simulink model "s_b8a4x128f"  (R2016b)
settings: Solver=VariableStepDiscrete  StartTime=0.0  StopTime=1  RelTol=1e-3
undefined symbols (not defined in the file): fft_stages, n_bits_ants, n_bits_xengs
libraries: xbsIndex_r4 x21069, casper_library_misc x164, casper_library_scopes x9, xbsReplacements_r4 x9, casper_library_delays x8, xps_library x3
(part 29 of 186)

== system s_b8a4x128f/sys1/x_cast ==
  in : Inport
  Concat : xbsIndex_r4/Concat  num_inputs=8  dbl_ovrd=off  block_type=concat
      settings: block_version=9.2.01
  Convert{,1..7} (8 alike) : xbsIndex_r4/Convert  gui_display_data_type=Fixed-point  arith_type="Signed  (2's comp)"  n_bits=n_bits_out  bin_pt=fix_pnt_pos  float_type=Single  exp_bits=8  fraction_bits=24  quantization=Truncate  overflow=Wrap  en=off  latency=0  pipeline=off  dbl_ovrd=off  block_type=convert
      settings: block_version=10.1.3
  Slice : xbsIndex_r4/Slice  nbits=n_bits_in  boolean_output=off  mode=Lower Bit Location + Width  bit1=0  base1=MSB of Input  bit0=bit_offsets(1)*n_bits_in  base0=LSB of Input  dbl_ovrd=off  block_type=slice
      settings: infoedit="Extracts a given range of bits from each input sample and presents it at the output.  The output type is ordinarily unsigned with binary point at zero, but can be Boolean when the slice is one bit wide.<P><P>Hardware notes: In hardware this block costs nothing."  block_version=10.1.3
  Slice1 : xbsIndex_r4/Slice  nbits=n_bits_in  boolean_output=off  mode=Lower Bit Location + Width  bit1=0  base1=MSB of Input  bit0=bit_offsets(2)*n_bits_in  base0=LSB of Input  dbl_ovrd=off  block_type=slice
      settings: infoedit="Extracts a given range of bits from each input sample and presents it at the output.  The output type is ordinarily unsigned with binary point at zero, but can be Boolean when the slice is one bit wide.<P><P>Hardware notes: In hardware this block costs nothing."  block_version=10.1.3
  Slice2 : xbsIndex_r4/Slice  nbits=n_bits_in  boolean_output=off  mode=Lower Bit Location + Width  bit1=0  base1=MSB of Input  bit0=bit_offsets(3)*n_bits_in  base0=LSB of Input  dbl_ovrd=off  block_type=slice
      settings: infoedit="Extracts a given range of bits from each input sample and presents it at the output.  The output type is ordinarily unsigned with binary point at zero, but can be Boolean when the slice is one bit wide.<P><P>Hardware notes: In hardware this block costs nothing."  block_version=10.1.3
  Slice3 : xbsIndex_r4/Slice  nbits=n_bits_in  boolean_output=off  mode=Lower Bit Location + Width  bit1=0  base1=MSB of Input  bit0=bit_offsets(4)*n_bits_in  base0=LSB of Input  dbl_ovrd=off  block_type=slice
      settings: infoedit="Extracts a given range of bits from each input sample and presents it at the output.  The output type is ordinarily unsigned with binary point at zero, but can be Boolean when the slice is one bit wide.<P><P>Hardware notes: In hardware this block costs nothing."  block_version=10.1.3
  Slice4 : xbsIndex_r4/Slice  nbits=n_bits_in  boolean_output=off  mode=Lower Bit Location + Width  bit1=0  base1=MSB of Input  bit0=bit_offsets(5)*n_bits_in  base0=LSB of Input  dbl_ovrd=off  block_type=slice
      settings: infoedit="Extracts a given range of bits from each input sample and presents it at the output.  The output type is ordinarily unsigned with binary point at zero, but can be Boolean when the slice is one bit wide.<P><P>Hardware notes: In hardware this block costs nothing."  block_version=10.1.3
  Slice5 : xbsIndex_r4/Slice  nbits=n_bits_in  boolean_output=off  mode=Lower Bit Location + Width  bit1=0  base1=MSB of Input  bit0=bit_offsets(6)*n_bits_in  base0=LSB of Input  dbl_ovrd=off  block_type=slice
      settings: infoedit="Extracts a given range of bits from each input sample and presents it at the output.  The output type is ordinarily unsigned with binary point at zero, but can be Boolean when the slice is one bit wide.<P><P>Hardware notes: In hardware this block costs nothing."  block_version=10.1.3
  Slice6 : xbsIndex_r4/Slice  nbits=n_bits_in  boolean_output=off  mode=Lower Bit Location + Width  bit1=0  base1=MSB of Input  bit0=bit_offsets(7)*n_bits_in  base0=LSB of Input  dbl_ovrd=off  block_type=slice
      settings: infoedit="Extracts a given range of bits from each input sample and presents it at the output.  The output type is ordinarily unsigned with binary point at zero, but can be Boolean when the slice is one bit wide.<P><P>Hardware notes: In hardware this block costs nothing."  block_version=10.1.3
  Slice7 : xbsIndex_r4/Slice  nbits=n_bits_in  boolean_output=off  mode=Lower Bit Location + Width  bit1=0  base1=MSB of Input  bit0=bit_offsets(8)*n_bits_in  base0=LSB of Input  dbl_ovrd=off  block_type=slice
      settings: infoedit="Extracts a given range of bits from each input sample and presents it at the output.  The output type is ordinarily unsigned with binary point at zero, but can be Boolean when the slice is one bit wide.<P><P>Hardware notes: In hardware this block costs nothing."  block_version=10.1.3
  force_re{,1,4,6,8,10,12,14} (8 alike) : xbsIndex_r4/Reinterpret  force_arith_type=on  arith_type="Signed  (2's comp)"  force_bin_pt=on  bin_pt=fix_pnt_pos  block_type=reinterpret
      settings: infoedit="Changes signal type without altering the binary representation.   You can changed the signal between signed and unsigned, and relocate the binary point.<P><P>Hardware notes: In hardware this block costs nothing.<P><P>Example:  Suppose the input is 6 bits wide, signed, with 2 fractional bits, and the output is forced to unsigned with 0 fractional bits.  Then an input of -2.0 (1110.00 in binary 2's complement) becomes an output of 56 (111000 in binary)."  block_version=9.1.01
  force_re{2..3,5,7,9,11,13,15} (8 alike) : xbsIndex_r4/Reinterpret  force_arith_type=on  arith_type=Unsigned  force_bin_pt=on  bin_pt=0  block_type=reinterpret
      settings: infoedit="Changes signal type without altering the binary representation.   You can changed the signal between signed and unsigned, and relocate the binary point.<P><P>Hardware notes: In hardware this block costs nothing.<P><P>Example:  Suppose the input is 6 bits wide, signed, with 2 fractional bits, and the output is forced to unsigned with 0 fractional bits.  Then an input of -2.0 (1110.00 in binary 2's complement) becomes an output of 56 (111000 in binary)."  block_version=9.1.01
  out : Outport
  wires:
  force_re2/1 -> Concat/1
  Convert/1 -> force_re2/1
  Convert1/1 -> force_re3/1
  force_re/1 -> Convert/1
  force_re1/1 -> Convert1/1
  Slice/1 -> force_re/1
  in/1 -> Slice/1, Slice6/1, Slice7/1, Slice5/1, Slice4/1, Slice3/1, Slice2/1, Slice1/1
  Concat/1 -> out/1
  Slice1/1 -> force_re1/1
  force_re3/1 -> Concat/2
  Convert2/1 -> force_re5/1
  force_re4/1 -> Convert2/1
  Slice2/1 -> force_re4/1
  Convert3/1 -> force_re7/1
  force_re6/1 -> Convert3/1
  Slice3/1 -> force_re6/1
  Convert4/1 -> force_re9/1
  force_re8/1 -> Convert4/1
  Slice4/1 -> force_re8/1
  Convert5/1 -> force_re11/1
  force_re10/1 -> Convert5/1
  Slice5/1 -> force_re10/1
  Convert6/1 -> force_re13/1
  force_re12/1 -> Convert6/1
  Slice6/1 -> force_re12/1
  Convert7/1 -> force_re15/1
  force_re14/1 -> Convert7/1
  Slice7/1 -> force_re14/1
  force_re5/1 -> Concat/3
  force_re7/1 -> Concat/4
  force_re9/1 -> Concat/5
  force_re11/1 -> Concat/6
  force_re13/1 -> Concat/7
  force_re15/1 -> Concat/8

== system s_b8a4x128f/sys1/xeng ==
  sync_in : Inport
  ant : Inport  Port=2
  window_valid : Inport  Port=3
  mcnt_in : Inport  Port=4
  Constant : xbsIndex_r4/Constant  const=0  gui_display_data_type=Fixed-point  arith_type=Unsigned  n_bits=200  bin_pt=14  preci_type=Single  exp_width=8  frac_width=24  explicit_period=on  period=1  equ=P=C  opselect=C  inp2=PCIN>>17  opr=+  inp1=P  carry=CIN  dbl_ovrd=off  block_type=constant
  Constant1 : xbsIndex_r4/Constant  const=0  gui_display_data_type=Fixed-point  arith_type=Boolean  n_bits=1  bin_pt=14  preci_type=Single  exp_width=8  frac_width=24  explicit_period=on  period=1  equ=P=C  opselect=C  inp2=PCIN>>17  opr=+  inp1=P  carry=CIN  dbl_ovrd=off  block_type=constant
  Term1 : Terminator
  Term2 : Terminator
  Term3 : Terminator
  auto_tap : Subsystem  AncestorBlock=casper_library_correlator/auto_tap  mask(auto_tap){n_ants=8, n_simultan=2, n_bits=8, acc_len=256, add_latency=3, mult_latency=4, bram_latency=7, mult_type=1, use_bram_delay=1}
      mask prompts: n_ants "Number of antennas (total inputs = n_ants*n_simultan below)"; n_simultan "Number of inputs fed-in simultaneously"; n_bits "Number of input bits (per complex component)"; acc_len "Accumulation length"; add_latency "Adder latency"; mult_latency "Multiplier latency"; bram_latency "BRAM latency"; mult_type "Multiplier Type (0=behavioural HDL, 1=embedded, 2=core)"; use_bram_delay "Implementation: Delay type (0=SLR, 1=BRAM)"
      mask init:
      | fix_pnt_pos = (n_bits-1)*2;
      | bit_growth = ceil(log2(acc_len));
      | ant_bits = ceil(log2(n_ants));
      | n_bits_out = (2*n_bits + 1 + bit_growth);
      | 
      | params = get_mask_params(gcb);
      | auto_tap_init(gcb, params{:});
      settings: AttributesFormatString=mult_typ=1, del_typ=1
  baseline_tap1 : Subsystem  AncestorBlock=casper_library_correlator/baseline_tap  mask(baseline_tap){n_ants=8, ant_sep=1, n_bits=8, acc_len=256, add_latency=3, mult_latency=4, bram_latency=7, mult_type=1, use_bram_delay=1}
      mask prompts: n_ants "Number of antennas"; ant_sep "Antenna Seperation"; n_bits "number of input bits (per complex component)"; acc_len "accumulation length"; add_latency "Adder latency"; mult_latency "Multiplier latency"; bram_latency "BRAM latency"; mult_type "Multiplier Type (0=behavioural HDL, 1=embedded, 2=core)"; use_bram_delay "Use BRAM delays"
      mask init: same as s_b8a4x128f/sys0/xeng/baseline_tap1
      settings: AttributesFormatString=ant_sep=1, mult=1, bram=1
  baseline_tap2 : Subsystem  AncestorBlock=casper_library_correlator/baseline_tap  mask(baseline_tap){n_ants=8, ant_sep=2, n_bits=8, acc_len=256, add_latency=3, mult_latency=4, bram_latency=7, mult_type=1, use_bram_delay=1}
      mask prompts: n_ants "Number of antennas"; ant_sep "Antenna Seperation"; n_bits "number of input bits (per complex component)"; acc_len "accumulation length"; add_latency "Adder latency"; mult_latency "Multiplier latency"; bram_latency "BRAM latency"; mult_type "Multiplier Type (0=behavioural HDL, 1=embedded, 2=core)"; use_bram_delay "Use BRAM delays"
      mask init: same as s_b8a4x128f/sys0/xeng/baseline_tap1
      settings: AttributesFormatString=ant_sep=2, mult=1, bram=1
  baseline_tap3 : Subsystem  AncestorBlock=casper_library_correlator/baseline_tap  mask(baseline_tap){n_ants=8, ant_sep=3, n_bits=8, acc_len=256, add_latency=3, mult_latency=4, bram_latency=7, mult_type=1, use_bram_delay=1}
      mask prompts: n_ants "Number of antennas"; ant_sep "Antenna Seperation"; n_bits "number of input bits (per complex component)"; acc_len "accumulation length"; add_latency "Adder latency"; mult_latency "Multiplier latency"; bram_latency "BRAM latency"; mult_type "Multiplier Type (0=behavioural HDL, 1=embedded, 2=core)"; use_bram_delay "Use BRAM delays"
      mask init: same as s_b8a4x128f/sys0/xeng/baseline_tap1
      settings: AttributesFormatString=ant_sep=3, mult=1, bram=1
  baseline_tap4 : Subsystem  AncestorBlock=casper_library_correlator/baseline_tap  mask(baseline_tap){n_ants=8, ant_sep=4, n_bits=8, acc_len=256, add_latency=3, mult_latency=4, bram_latency=7, mult_type=1, use_bram_delay=1}
      mask prompts: n_ants "Number of antennas"; ant_sep "Antenna Seperation"; n_bits "number of input bits (per complex component)"; acc_len "accumulation length"; add_latency "Adder latency"; mult_latency "Multiplier latency"; bram_latency "BRAM latency"; mult_type "Multiplier Type (0=behavioural HDL, 1=embedded, 2=core)"; use_bram_delay "Use BRAM delays"
      mask init: same as s_b8a4x128f/sys0/xeng/baseline_tap1
      settings: AttributesFormatString=ant_sep=4, mult=1, bram=1
  delay : xbsIndex_r4/Delay  rst=off  infoeditControl=Selection of Reset will increase slice count due to use of real FFs and instead of SRLs  en=off  latency=1  reg_retiming=on  dbl_ovrd=off  block_type=delay
  sample_and_hold1 : Subsystem  AncestorBlock=casper_library_misc/sample_and_hold  mask(sample_and_hold){period=2048}
      mask prompts: period "Sample period (clocks)"
      mask help: This block will sample an input signal at a user specified rate and hold the value on the output.
  sample_and_hold2 : Subsystem  AncestorBlock=casper_library_misc/sample_and_hold  mask(sample_and_hold){period=2048}
      mask prompts: period "Sample period (clocks)"
      mask help: This block will sample an input signal at a user specified rate and hold the value on the output.
  sample_and_hold3 : Subsystem  AncestorBlock=casper_library_misc/sample_and_hold  mask(sample_and_hold){period=2048}
      mask prompts: period "Sample period (clocks)"
      mask help: This block will sample an input signal at a user specified rate and hold the value on the output.
  window_delay : casper_library_delays/window_delay  delay=269
  xeng_descramble : Subsystem  AncestorBlock=casper_library_correlator/xeng_descramble  mask(xeng_descramble){num_ants=8, n_bits=8, acc_len=256, demux_factor=1}
      mask prompts: num_ants "Number of Antennas"; n_bits "Input Bitwidth"; acc_len "X engine accumulation length"; demux_factor "Demux Factor"
      mask help:
      | NOT TESTED FOR non-2^N antennas.
      |
      | Descrambles X engine output. Optionally demuxes output.
      mask init: same as s_b8a4x128f/sys0/xeng/xeng_descramble
      settings: AttributesFormatString=num_ants=8
  sync_out : Outport
  valid : Outport  Port=2
  acc : Outport  Port=3
  mcnt_out : Outport  Port=4
  wires:
  xeng_descramble/1(acc_out) -> acc/1
  xeng_descramble/2(valid_out) -> valid/1
  xeng_descramble/3(sync_out) -> sync_out/1, sample_and_hold3/1(sync)
  baseline_tap4/4(acc_out) -> xeng_descramble/1(acc)
  baseline_tap4/5(valid_out) -> xeng_descramble/2(valid)
  baseline_tap4/7(sync_out) -> xeng_descramble/3(sync), sample_and_hold2/1(sync)
  window_delay/1 -> xeng_descramble/4(win_valid)
  ant/1 -> auto_tap/1(a_del), auto_tap/2(a_ndel)
  Constant/1 -> auto_tap/4(acc_in)
  Constant1/1 -> auto_tap/5(valid_in)
  sync_in/1 -> auto_tap/6(sync_in), sample_and_hold1/1(sync)
  window_valid/1 -> window_delay/1
  mcnt_in/1 -> sample_and_hold1/2(in)
  sample_and_hold1/1(out) -> sample_and_hold2/2(in)
  sample_and_hold2/1(out) -> sample_and_hold3/2(in)
  sample_and_hold3/1(out) -> delay/1
  delay/1 -> mcnt_out/1
  auto_tap/1(a_del_out) -> baseline_tap1/1(a_del)
  auto_tap/2(a_ndel_out) -> baseline_tap1/2(a_ndel)
  auto_tap/3(a_end_out) -> baseline_tap1/3(a_end)
  auto_tap/4(acc_out) -> baseline_tap1/4(acc_in)
  auto_tap/5(valid_out) -> baseline_tap1/5(valid_in)
  auto_tap/6(rst_out) -> baseline_tap1/6(rst)
  auto_tap/7(sync_out) -> baseline_tap1/7(sync1)
  baseline_tap1/1(a_del_out) -> baseline_tap2/1(a_del)
  baseline_tap1/2(a_ndel_out) -> baseline_tap2/2(a_ndel)
  baseline_tap1/3(a_end_out) -> baseline_tap2/3(a_end)
  baseline_tap1/4(acc_out) -> baseline_tap2/4(acc_in)
  baseline_tap1/5(valid_out) -> baseline_tap2/5(valid_in)
  baseline_tap1/6(rst_out) -> baseline_tap2/6(rst)
  baseline_tap1/7(sync_out) -> baseline_tap2/7(sync1)
  baseline_tap2/1(a_del_out) -> baseline_tap3/1(a_del)
  baseline_tap2/2(a_ndel_out) -> baseline_tap3/2(a_ndel)
  baseline_tap2/3(a_end_out) -> baseline_tap3/3(a_end)
  baseline_tap2/4(acc_out) -> baseline_tap3/4(acc_in)
  baseline_tap2/5(valid_out) -> baseline_tap3/5(valid_in)
  baseline_tap2/6(rst_out) -> baseline_tap3/6(rst)
  baseline_tap2/7(sync_out) -> baseline_tap3/7(sync1)
  baseline_tap3/1(a_del_out) -> baseline_tap4/1(a_del)
  baseline_tap3/2(a_ndel_out) -> baseline_tap4/2(a_ndel)
  baseline_tap3/3(a_end_out) -> baseline_tap4/3(a_end)
  baseline_tap3/4(acc_out) -> baseline_tap4/4(acc_in)
  baseline_tap3/5(valid_out) -> baseline_tap4/5(valid_in)
  baseline_tap3/6(rst_out) -> baseline_tap4/6(rst)
  baseline_tap3/7(sync_out) -> baseline_tap4/7(sync1)
  baseline_tap4/1(a_del_out) -> auto_tap/3(a_loop)
  baseline_tap4/2(a_ndel_out) -> Term1/1
  baseline_tap4/3(a_end_out) -> Term2/1
  baseline_tap4/6(rst_out) -> Term3/1

== system s_b8a4x128f/sys1/xeng_pack_out ==
  note: we must create a gap
      | between packets from
      | mutliple x-engines to allow
      | the buffers on the output switch
      | ports to drain and NIC card
      | to service the packets.
  note: if we become misaligned,
      | then we must flush the buffers
      | by reading one word, waiting "fifo_latency" clocks,
      | then reading another word until we get rb_done.
  note: the last packet
      | might be shorter!
  data_in : Inport
  valid_in : Inport  Port=2
  pkt_rdy : Inport  Port=3
  rb_done : Inport  Port=4
  timestamp : Inport  Port=5
  xeng_id : Inport  Port=6
  go : Inport  Port=7
  gap_size : Inport  Port=8
  AddSub1 : xbsIndex_r4/AddSub  mode=Subtraction  use_carryin=off  use_carryout=off  en=off  latency=1  precision=User Defined  arith_type=Unsigned  n_bits=vector_bits+1  bin_pt=0  quantization=Truncate  overflow=Saturate  use_behavioral_HDL=on  hw_selection=Fabric  pipelined=off  dbl_ovrd=off  block_type=addsub
  Concat : xbsIndex_r4/Concat  num_inputs=2  dbl_ovrd=off  block_type=concat
  Constant : xbsIndex_r4/Constant  const=0  gui_display_data_type=Boolean  arith_type=Boolean  n_bits=16  bin_pt=14  preci_type=Single  exp_width=8  frac_width=24  explicit_period=on  period=1  equ=P=C  opselect=C  inp2=PCIN>>17  opr=+  inp1=P  carry=CIN  dbl_ovrd=off  block_type=constant
  Constant1 : xbsIndex_r4/Constant  const=0  gui_display_data_type=Fixed-point  arith_type=Unsigned  n_bits=spead_lsw  bin_pt=0  preci_type=Single  exp_width=8  frac_width=24  explicit_period=on  period=1  equ=P=C  opselect=C  inp2=PCIN>>17  opr=+  inp1=P  carry=CIN  dbl_ovrd=off  block_type=constant
  Constant15 : xbsIndex_r4/Constant  const=pkt_len  gui_display_data_type=Fixed-point  arith_type=Unsigned  n_bits=vector_bits+1  bin_pt=0  preci_type=Single  exp_width=8  frac_width=24  explicit_period=on  period=1  equ=P=C  opselect=C  inp2=PCIN>>17  opr=+  inp1=P  carry=CIN  dbl_ovrd=off  block_type=constant
  Constant2 : xbsIndex_r4/Constant  const=(vector_len)-1  gui_display_data_type=Fixed-point  arith_type=Unsigned  n_bits=vector_bits+1  bin_pt=0  preci_type=Single  exp_width=8  frac_width=24  explicit_period=on  period=1  equ=P=C  opselect=C  inp2=PCIN>>17  opr=+  inp1=P  carry=CIN  dbl_ovrd=off  block_type=constant
  Constant3 : xbsIndex_r4/Constant  const=vector_len  gui_display_data_type=Fixed-point  arith_type=Unsigned  n_bits=vector_bits+1  bin_pt=0  preci_type=Single  exp_width=8  frac_width=24  explicit_period=on  period=1  equ=P=C  opselect=C  inp2=PCIN>>17  opr=+  inp1=P  carry=CIN  dbl_ovrd=off  block_type=constant
  Constant4 : xbsIndex_r4/Constant  const=0  gui_display_data_type=Boolean  arith_type=Boolean  n_bits=16  bin_pt=14  preci_type=Single  exp_width=8  frac_width=24  explicit_period=on  period=1  equ=P=C  opselect=C  inp2=PCIN>>17  opr=+  inp1=P  carry=CIN  dbl_ovrd=off  block_type=constant
  Constant6 : xbsIndex_r4/Constant  const=heap_len  gui_display_data_type=Fixed-point  arith_type=Unsigned  n_bits=spead_lsw  bin_pt=0  preci_type=Single  exp_width=8  frac_width=24  explicit_period=on  period=1  equ=P=C  opselect=C  inp2=PCIN>>17  opr=+  inp1=P  carry=CIN  dbl_ovrd=off  block_type=constant
  Constant7 : xbsIndex_r4/Constant  const=pkt_len-1  gui_display_data_type=Fixed-point  arith_type=Unsigned  n_bits=pkt_bits  bin_pt=0  preci_type=Single  exp_width=8  frac_width=24  explicit_period=on  period=1  equ=P=C  opselect=C  inp2=PCIN>>17  opr=+  inp1=P  carry=CIN  dbl_ovrd=off  block_type=constant
  Constant8 : xbsIndex_r4/Constant  const=1  gui_display_data_type=Fixed-point  arith_type=Unsigned  n_bits=ceil(log2(fifo_latency))+1  bin_pt=0  preci_type=Single  exp_width=8  frac_width=24  explicit_period=on  period=1  equ=P=C  opselect=C  inp2=PCIN>>17  opr=+  inp1=P  carry=CIN  dbl_ovrd=off  block_type=constant
  Convert{,1..4,6} (6 alike) : xbsIndex_r4/Convert  gui_display_data_type=Fixed-point  arith_type=Unsigned  n_bits=spead_lsw  bin_pt=0  float_type=Single  exp_bits=8  fraction_bits=24  quantization=Truncate  overflow=Wrap  en=off  latency=0  pipeline=off  dbl_ovrd=off  block_type=convert
      settings: block_version=11.4
  Counter1 : xbsIndex_r4/Counter  cnt_type=Free Running  cnt_to=1023  operation=Up  start_count=0  cnt_by_val=1  arith_type=Unsigned  n_bits=vector_bits+1  bin_pt=0  load_pin=off  rst=on  en=on  explicit_period=on  period=1  use_behavioral_HDL=off  implementation=Fabric  use_rpm=on  dbl_ovrd=off  block_type=counter
      settings: xl_area=[0, 0, 0, 0, 0, 0, 0]
  Delay{,3,6,10..17} (11 alike) : xbsIndex_r4/Delay  rst=off  infoeditControl=Selection of Reset will increase slice count due to use of real FFs and instead of SRLs  en=off  latency=1  reg_retiming=on  dbl_ovrd=off  block_type=delay
      settings: block_version=11.4
  Delay1 : xbsIndex_r4/Delay  rst=off  infoeditControl=Selection of Reset will increase slice count due to use of real FFs and instead of SRLs  en=on  latency=1  reg_retiming=on  dbl_ovrd=off  block_type=delay
  Delay2 : xbsIndex_r4/Delay  rst=off  infoeditControl=Selection of Reset will increase slice count due to use of real FFs and instead of SRLs  en=off  latency=fifo_latency  reg_retiming=on  dbl_ovrd=off  block_type=delay
      settings: block_version=11.4
  Delay4 : xbsIndex_r4/Delay  rst=off  infoeditControl=Selection of Reset will increase slice count due to use of real FFs and instead of SRLs  en=off  latency=fifo_latency  reg_retiming=on  dbl_ovrd=off  block_type=delay
      settings: block_version=11.4
  Delay5 : xbsIndex_r4/Delay  rst=off  infoeditControl=Selection of Reset will increase slice count due to use of real FFs and instead of SRLs  en=on  latency=1  reg_retiming=on  dbl_ovrd=off  block_type=delay
  Delay7 : xbsIndex_r4/Delay  rst=on  infoeditControl=Selection of Reset will increase slice count due to use of real FFs and instead of SRLs  en=on  latency=1  reg_retiming=on  dbl_ovrd=off  block_type=delay
  Delay8 : xbsIndex_r4/Delay  rst=on  infoeditControl=Selection of Reset will increase slice count due to use of real FFs and instead of SRLs  en=on  latency=1  reg_retiming=on  dbl_ovrd=off  block_type=delay
  Delay9 : xbsIndex_r4/Delay  rst=on  infoeditControl=Selection of Reset will increase slice count due to use of real FFs and instead of SRLs  en=on  latency=1  reg_retiming=on  dbl_ovrd=off  block_type=delay
  Gateway Out{1..21} (21 alike) : xbsIndex_r4/Gateway Out  inherit_from_input=off  hdl_port=off  rows=1  columns=1  UseAsDAC=off  DACChannel='1'  interface=None  automatic_assignment=on  address_offset=hex2dec('00')  intf_name=''  intf_description=''  timing_constraint=None  locs_specified=off  LOCs={}  io_standard={}  block_type=gatewayout
      settings: xl_area=[0, 0, 0, 0, 0, 0, 0]  block_version=10.1.3
  Inverter{1..4} (4 alike) : xbsIndex_r4/Inverter  en=off  latency=0  dbl_ovrd=off  block_type=inv
      settings: block_version=11.4
  Logical{1,3..5,13..14} (6 alike) : xbsIndex_r4/Logical  logical_function=OR  inputs=2  en=off  latency=0  precision=Full  arith_type=Unsigned  n_bits=8  bin_pt=2  align_bp=on  dbl_ovrd=off  block_type=logical
      settings: xl_area=[0, 0, 0, 0, 0, 0, 0]
  Logical{2,8..12,15} (7 alike) : xbsIndex_r4/Logical  logical_function=AND  inputs=2  en=off  latency=0  precision=Full  arith_type=Unsigned  n_bits=8  bin_pt=2  align_bp=on  dbl_ovrd=off  block_type=logical
      settings: xl_area=[0, 0, 0, 0, 0, 0, 0]
  Logical6 : xbsIndex_r4/Logical  logical_function=AND  inputs=2  en=off  latency=1  precision=Full  arith_type=Unsigned  n_bits=8  bin_pt=2  align_bp=on  dbl_ovrd=off  block_type=logical
      settings: xl_area=[0, 0, 0, 0, 0, 0, 0]
  Logical7 : xbsIndex_r4/Logical  logical_function=XOR  inputs=2  en=off  latency=0  precision=Full  arith_type=Unsigned  n_bits=8  bin_pt=2  align_bp=on  dbl_ovrd=off  block_type=logical
      settings: xl_area=[0, 0, 0, 0, 0, 0, 0]
  Mux1 : xbsIndex_r4/Mux  inputs=2  en=off  latency=1  precision=Full  arith_type="Signed  (2's comp)"  n_bits=8  bin_pt=2  quantization=Truncate  overflow=Wrap  dbl_ovrd=off  block_type=mux
      settings: xl_area=[0, 0, 0, 0, 0, 0, 0]
  Reinterpret : xbsIndex_r4/Reinterpret  force_arith_type=on  arith_type=Unsigned  force_bin_pt=on  bin_pt=0  block_type=reinterpret
      settings: infoedit="Changes signal type without altering the binary representation.   You can changed the signal between signed and unsigned, and relocate the binary point.<br><br>Hardware notes: In hardware this block costs nothing.<br><br>Example:  Suppose the input is 6 bits wide, signed, with 2 fractional bits, and the output is forced to unsigned with 0 fractional bits.  Then an input of -2.0 (1110.00 in binary 2's complement) becomes an output of 56 (111000 in binary)."
  Relational1 : xbsIndex_r4/Relational  mode=a=b  op_type=Bool  en=off  latency=0  dbl_ovrd=off  block_type=relational
      settings: xl_area=[0, 0, 0, 0, 0, 0, 0]  block_version=10.1.3
  Relational2 : xbsIndex_r4/Relational  mode=a<b  op_type=Bool  en=off  latency=0  dbl_ovrd=off  block_type=relational
      settings: xl_area=[0, 0, 0, 0, 0, 0, 0]  block_version=10.1.3
  Relational4 : xbsIndex_r4/Relational  mode=a=b  op_type=Bool  en=off  latency=0  dbl_ovrd=off  block_type=relational
      settings: xl_area=[0, 0, 0, 0, 0, 0, 0]  block_version=10.1.3
  Relational5 : xbsIndex_r4/Relational  mode=a=b  op_type=Bool  en=off  latency=0  dbl_ovrd=off  block_type=relational
      settings: xl_area=[0, 0, 0, 0, 0, 0, 0]  block_version=10.1.3
  Shift1 : xbsIndex_r4/Shift  shift_dir=Left  shift_bits=n_bits_word_size  en=off  latency=0  precision=Full  arith_type="Signed  (2's comp)"  n_bits=16  bin_pt=14  quantization=Truncate  overflow=Wrap  dbl_ovrd=off  block_type=shift
  Shift2 : xbsIndex_r4/Shift  shift_dir=Left  shift_bits=n_bits_chans  en=off  latency=0  precision=Full  arith_type="Signed  (2's comp)"  n_bits=16  bin_pt=14  quantization=Truncate  overflow=Wrap  dbl_ovrd=off  block_type=shift
  Slice : xbsIndex_r4/Slice  nbits=pkt_bits  boolean_output=off  mode=Lower Bit Location + Width  bit1=0  base1=MSB of Input  bit0=0  base0=LSB of Input  dbl_ovrd=off  block_type=slice
  Slice1 : xbsIndex_r4/Slice  nbits=1  boolean_output=off  mode=Two Bit Locations  bit1=0  base1=MSB of Input  bit0=n_bits_timestamp_padding  base0=LSB of Input  dbl_ovrd=off  block_type=slice
  edge_detect : Subsystem  AncestorBlock=casper_library_misc/edge_detect  mask(edge_detect){edge=Rising, polarity=Active High, x_in=[0 0.08 0.08 0.16 0.16 0.24 0.24 0.32 0.32 0.4], y_in=[-1 -1  1  1  1  1  1  1  1  1], x_out=[0.6 0.68 0.68 0.76 0.76 0.84 0.84 0.92 0.92 1], y_out=[-1 -1  1  1 -1 -1 -1 -1 -1 -1]}
      mask prompts: edge "Edge Type"; polarity "Output Polarity"; x_in "Input X Positions"; y_in "Input Y Positions"; x_out "Output X Positions"; y_out "Output Y Positions"
      mask help: Output is active for one-cycle after each edge of the specified type (i.e. rising, falling or both).
      mask init: same as s_b8a4x128f/edge_detect
      settings: AttributesFormatString=|
      | rising edges
      | active high
      mask Help: Output is active for one-cycle after each edge of the specified type (i.e. rising, falling, or both).  Latency is zero.
      mask TypeOptions edge: Rising | Falling | Both
      mask TypeOptions polarity: Active High | Active Low
      mask Display:
      | plot(x_in_num,0.5+y_in_num*0.2);
      | plot(x_out_num,0.5+y_out_num*0.2);
  edge_detect1 : Subsystem  AncestorBlock=casper_library_misc/edge_detect  mask(edge_detect){edge=Rising, polarity=Active High, x_in=[0 0.08 0.08 0.16 0.16 0.24 0.24 0.32 0.32 0.4], y_in=[-1 -1  1  1  1  1  1  1  1  1], x_out=[0.6 0.68 0.68 0.76 0.76 0.84 0.84 0.92 0.92 1], y_out=[-1 -1  1  1 -1 -1 -1 -1 -1 -1]}
      mask prompts: edge "Edge Type"; polarity "Output Polarity"; x_in "Input X Positions"; y_in "Input Y Positions"; x_out "Output X Positions"; y_out "Output Y Positions"
      mask help: Output is active for one-cycle after each edge of the specified type (i.e. rising, falling or both).
      mask init: same as s_b8a4x128f/edge_detect
      settings: AttributesFormatString=|
      | rising edges
      | active high
      mask Help: Output is active for one-cycle after each edge of the specified type (i.e. rising, falling, or both).  Latency is zero.
      mask TypeOptions edge: Rising | Falling | Both
      mask TypeOptions polarity: Active High | Active Low
      mask Display:
      | plot(x_in_num,0.5+y_in_num*0.2);
      | plot(x_out_num,0.5+y_out_num*0.2);
  edge_detect2 : Subsystem  AncestorBlock=casper_library_misc/edge_detect  mask(edge_detect){edge=Rising, polarity=Active High, x_in=[0 0.08 0.08 0.16 0.16 0.24 0.24 0.32 0.32 0.4], y_in=[-1 -1  1  1  1  1  1  1  1  1], x_out=[0.6 0.68 0.68 0.76 0.76 0.84 0.84 0.92 0.92 1], y_out=[-1 -1  1  1 -1 -1 -1 -1 -1 -1]}
      mask prompts: edge "Edge Type"; polarity "Output Polarity"; x_in "Input X Positions"; y_in "Input Y Positions"; x_out "Output X Positions"; y_out "Output Y Positions"
      mask help: Output is active for one-cycle after each edge of the specified type (i.e. rising, falling or both).
      mask init: same as s_b8a4x128f/edge_detect
      settings: AttributesFormatString=|
      | rising edges
      | active high
      mask Help: Output is active for one-cycle after each edge of the specified type (i.e. rising, falling, or both).  Latency is zero.
      mask TypeOptions edge: Rising | Falling | Both
      mask TypeOptions polarity: Active High | Active Low
      mask Display:
      | plot(x_in_num,0.5+y_in_num*0.2);
      | plot(x_out_num,0.5+y_out_num*0.2);
  edge_detect3 : Subsystem  AncestorBlock=casper_library_misc/edge_detect  mask(edge_detect){edge=Rising, polarity=Active High, x_in=[0 0.08 0.08 0.16 0.16 0.24 0.24 0.32 0.32 0.4], y_in=[-1 -1  1  1  1  1  1  1  1  1], x_out=[0.6 0.68 0.68 0.76 0.76 0.84 0.84 0.92 0.92 1], y_out=[-1 -1  1  1 -1 -1 -1 -1 -1 -1]}
      mask prompts: edge "Edge Type"; polarity "Output Polarity"; x_in "Input X Positions"; y_in "Input Y Positions"; x_out "Output X Positions"; y_out "Output Y Positions"
      mask help: Output is active for one-cycle after each edge of the specified type (i.e. rising, falling or both).
      mask init: same as s_b8a4x128f/edge_detect
      settings: AttributesFormatString=|
      | rising edges
      | active high
      mask Help: Output is active for one-cycle after each edge of the specified type (i.e. rising, falling, or both).  Latency is zero.
      mask TypeOptions edge: Rising | Falling | Both
      mask TypeOptions polarity: Active High | Active Low
      mask Display:
      | plot(x_in_num,0.5+y_in_num*0.2);
      | plot(x_out_num,0.5+y_out_num*0.2);
  edge_detect4 : Subsystem  AncestorBlock=casper_library_misc/edge_detect  mask(edge_detect){edge=Rising, polarity=Active High, x_in=[0 0.08 0.08 0.16 0.16 0.24 0.24 0.32 0.32 0.4], y_in=[-1 -1  1  1  1  1  1  1  1  1], x_out=[0.6 0.68 0.68 0.76 0.76 0.84 0.84 0.92 0.92 1], y_out=[-1 -1  1  1 -1 -1 -1 -1 -1 -1]}
      mask prompts: edge "Edge Type"; polarity "Output Polarity"; x_in "Input X Positions"; y_in "Input Y Positions"; x_out "Output X Positions"; y_out "Output Y Positions"
      mask help: Output is active for one-cycle after each edge of the specified type (i.e. rising, falling or both).
      mask init: same as s_b8a4x128f/edge_detect
      settings: AttributesFormatString=|
      | rising edges
      | active high
      mask Help: Output is active for one-cycle after each edge of the specified type (i.e. rising, falling, or both).  Latency is zero.
      mask TypeOptions edge: Rising | Falling | Both
      mask TypeOptions polarity: Active High | Active Low
      mask Display:
      | plot(x_in_num,0.5+y_in_num*0.2);
      | plot(x_out_num,0.5+y_out_num*0.2);
  gap_creator : xbsIndex_r4/Counter  cnt_type=Free Running  cnt_to=Inf  operation=Up  start_count=0  cnt_by_val=1  arith_type=Unsigned  n_bits=n_bits_max_gap  bin_pt=0  load_pin=off  rst=on  en=on  explicit_period=on  period=1  use_behavioral_HDL=off  implementation=Fabric  dbl_ovrd=off  block_type=counter
  gap_done : xbsIndex_r4/Relational  mode=a<b  op_type=Bool  en=off  latency=1  dbl_ovrd=off  block_type=relational
  hdr_check : Scope  NumInputPorts=5
  hdr_check1 : Scope  NumInputPorts=5
  pack_xeng : Subsystem  Tag=casper:spead_pack  AncestorBlock=casper_library_communications/spead_pack  mask(pkt_pack_mask){max_pkt_len_bits=8, header_ids=0x1600, 0x4103, header_ind_ids=0x1800, spead_msw=64, spead_lsw=48, spead_version=4, bytes_per_word=8}
      mask prompts: max_pkt_len_bits "Max pkt length, 2^? 64-bit words"; header_ids "SPEAD direct address IDs (decimal)"; header_ind_ids "SPEAD indirect address IDs (decimal)"; spead_msw "SPEAD Flavour (MSw)"; spead_lsw "SPEAD Flavour (LSw)"; spead_version "SPEAD version"; bytes_per_word "Word size, in bytes"
      mask help:
      | This block generates SPEAD-compliant packets from a datastream.
      |
      | Packets are created with a fixed header followed by a number of 64-bit items.
      |
      | Requires a 64-bit data stream.
      |
      | The data_ready signal is one cycle BEFORE valid data! Does not have to be with a valid signal either.
      mask init:
      | % if floor(log2(bytes_per_word)) ~= log2(bytes_per_word)
      | %     error('Bytes per word should be a power of two.');
      | % end
      | % 
      | % spead_pack_init(gcb)
  packetise_output : Scope  NumInputPorts=11
  payload_cnt4 : xbsIndex_r4/Counter  cnt_type=Count Limited  cnt_to=max((fifo_latency + 1),2)  operation=Up  start_count=0  cnt_by_val=1  arith_type=Unsigned  n_bits=ceil(log2(fifo_latency))+1  bin_pt=0  load_pin=off  rst=on  en=on  explicit_period=on  period=1  use_behavioral_HDL=off  implementation=Fabric  use_rpm=on  dbl_ovrd=off  block_type=counter
      settings: xl_area=[0, 0, 0, 0, 0, 0, 0]
  status : Subsystem  Tag=xps:sw_reg  AncestorBlock=xps_library/software register  mask(swreg){io_dir=To Processor, io_delay=1, sample_period=1, names=[pkt_cnt align_err_cnt overflow_err_cnt], bitwidths=[16 8 8], bin_pts=0, arith_types=0, sim_port=off, show_format=off}
      mask prompts: io_dir "I/O direction"; io_delay "I/O delay"; sample_period "Sample period"; names "Bitfield names [msb...lsb]"; bitwidths "Bitfield widths"; bin_pts "Bitfield binary pts"; arith_types "Bitfield types, ufix=0, fix=1, bool=2"; sim_port "Provide sim input/output?"; show_format "Print format string?"
      mask help: A 32-bit software-accessible register. Can be divided into bitfields of varying widths and types using the fields in the block mask.
      mask init:
      | try
      |     swreg_init(gcb)
      | catch ex
      |     disp(sprintf('%s: %s', gcb, ex.message))
      |     errordlg(ex.message)
      | end
      settings: AttributesFormatString=3 outputs
      mask TypeOptions io_dir: To Processor | From Processor
      mask Callback io_dir:
      | mask_enables = get_param(gcb, 'MaskEnables');
      | mask_names = get_param(gcb, 'MaskNames');
      | if strcmp(get_param(gcb, 'io_dir'), 'To Processor'),
      |     mask_enables{ismember(mask_names, 'sample_period')} = 'off';
      | else
      |     mask_enables{ismember(mask_names, 'sample_period')} = 'on';
      | end
      | set_param(gcb, 'MaskEnables', mask_enables);
  vacc_monitor3 : Subsystem
  data_out : Outport
  valid_out : Outport  Port=2
  eof : Outport  Port=3
  err : Outport  Port=4
  fetch : Outport  Port=5
  pkt_ready : Outport  Port=6
  wires:
  edge_detect4/1(out) -> gap_creator/1
  Convert6/1 -> Shift2/1
  Constant1/1 -> pack_xeng/10(hdr8_0x1800)
  Convert2/1 -> [heap_cnt]
  Concat/1 -> Convert2/1
  [xeng_id] -> Concat/2
  Slice1/1 -> Concat/1
  [timestamp] -> Slice1/1
  gap_size/1 -> [gap_size]
  Delay13/1 -> pack_xeng/9(hdr6_0x4103_DIR)
  [freq_offset] -> Delay13/1
  Shift2/1 -> [freq_offset]
  [xeng_id] -> Convert6/1
  Convert4/1 -> Delay16/1
  [gap_size] -> gap_done/2
  pack_xeng/3(eof) -> Logical3/1
  Logical3/1 -> [eof_out], eof/1
  Gateway Out15/1 -> packetise_output/7
  [end_of_vector] -> Logical5/1
  Gateway Out9/1 -> packetise_output/6
  Gateway Out14/1 -> packetise_output/5
  Gateway Out6/1 -> packetise_output/4
  Gateway Out8/1 -> packetise_output/3
  Gateway Out1/1 -> packetise_output/2
  Gateway Out7/1 -> packetise_output/1
  Logical5/1 -> [eof]
  Logical2/1 -> [rb_done]
  xeng_id/1 -> [xeng_id]
  Reinterpret/1 -> [data_input]
  Gateway Out11/1 -> packetise_output/8
  Slice/1 -> Relational1/1
  Counter1/1 -> [vector_position], Slice/1, Relational5/1
  timestamp/1 -> Delay5/1
  Delay5/1 -> [timestamp]
  [vector_start] -> Delay5/2
  Constant2/1 -> Relational5/2
  Relational5/1 -> [end_of_vector]
  data_in/1 -> Reinterpret/1, [raw_data_input]
  valid_in/1 -> Logical2/1, [valid_input]
  pkt_rdy/1 -> [pkt_rdy]
  rb_done/1 -> Logical2/2
  Gateway Out18/1 -> packetise_output/9
  Gateway Out17/1 -> packetise_output/10
  [valid_input] -> [valid_output]
  [fetch_pld] -> Counter1/2
  [vector_start] -> Counter1/1
  Constant7/1 -> Relational1/2
  Relational1/1 -> Logical5/2
  [fetch_pld] -> Gateway Out6/1
  [busy] -> Gateway Out15/1
  [valid_output] -> Gateway Out1/1
  [busy_pkt] -> Gateway Out9/1
  [raw_data_input] -> Gateway Out7/1
  [vector_position] -> Gateway Out11/1
  pack_xeng/1(data_out) -> data_out/1, [data_out]
  [vector_position] -> Delay1/1
  Delay1/1 -> AddSub1/2, Delay17/1
  [get_a_pkt] -> Delay1/2
  [rb_done] -> Logical7/1
  [end_of_vector] -> Delay2/1
  Delay17/1 -> Convert/1
  Convert/1 -> Shift1/1
  [vector_start] -> Logical4/1
  Logical4/1 -> Delay4/1
  [go] -> Logical8/1
  Logical8/1 -> Delay3/1
  Delay7/1 -> [busy], edge_detect/1(in)
  edge_detect/1(out) -> [vector_start]
  Inverter2/1 -> Logical10/1
  Logical10/1 -> Delay7/1, Delay7/3
  [end_of_vector] -> Logical1/2
  [go] -> Delay/1
  edge_detect1/1(out) -> Logical10/2
  [busy] -> Inverter2/1
  Delay/1 -> edge_detect1/1(in)
  Delay2/1 -> Logical7/2
  [get_a_pkt] -> Inverter1/1
  Delay3/1 -> Logical4/2
  Delay4/1 -> Delay8/1, Delay8/3
  edge_detect2/1(out) -> [get_a_pkt]
  Delay8/1 -> [busy_pkt], edge_detect2/1(in)
  [eof] -> Delay8/2
  [busy] -> Logical8/2
  Inverter1/1 -> Logical9/1
  Logical9/1 -> [fetch_pld]
  [eof] -> Gateway Out18/1
  [pkt_rdy] -> Gateway Out17/1
  Logical7/1 -> Delay9/1, Delay9/3, [err]
  [rb_done] -> Logical12/2
  payload_cnt4/1 -> Relational4/2
  Constant8/1 -> Relational4/1
  Delay9/1 -> payload_cnt4/2, [flushing]
  Relational4/1 -> [stutter_flush]
  Logical1/1 -> Delay7/2
  [err] -> Logical1/1
  [valid_output] -> Logical11/1
  Inverter3/1 -> Logical11/2, Logical15/2
  [flushing] -> Inverter3/1
  Logical12/1 -> Delay9/2, payload_cnt4/1
  [flushing] -> Logical12/1
  Logical13/1 -> fetch/1
  [fetch_pld] -> Logical13/1
  [stutter_flush] -> Logical13/2
  [data_out] -> Gateway Out2/1
  [vector_start] -> Gateway Out3/1
  [heap_cnt] -> Gateway Out4/1
  [heap_offset] -> Gateway Out5/1
  Gateway Out2/1 -> hdr_check/1
  Gateway Out3/1 -> hdr_check/2
  Gateway Out4/1 -> hdr_check/3
  Gateway Out5/1 -> hdr_check/4
  Constant15/1 -> Relational2/2, Mux1/2
  Mux1/1 -> Convert1/1
  Relational2/1 -> Mux1/1
  Constant3/1 -> AddSub1/1
  AddSub1/1 -> Mux1/3, Relational2/1
  Convert1/1 -> [pld_len]
  Shift1/1 -> [heap_offset]
  Gateway Out10/1 -> hdr_check/5
  [pld_len] -> Gateway Out10/1
  gap_creator/1 -> gap_done/1, [gap_count]
  go/1 -> [go]
  gap_done/1 -> Inverter4/1, gap_creator/2
  Inverter4/1 -> Logical6/1
  [pkt_rdy] -> Logical6/2
  Logical6/1 -> pkt_ready/1
  [eof] -> Delay6/1
  Gateway Out16/1 -> packetise_output/11
  [gap_count] -> Gateway Out16/1
  [data_input] -> Delay11/1
  [heap_cnt] -> Convert3/1
  [heap_offset] -> Delay14/1
  Logical11/1 -> Delay10/1
  pack_xeng/2(valid_out) -> valid_out/1
  [pld_len] -> Delay15/1
  Logical14/1 -> Logical3/2, err/1
  pack_xeng/4(data_overflow) -> [data_overflow], Logical14/2
  [err] -> Logical14/1
  [valid_output] -> Logical15/1
  edge_detect3/1(out) -> pack_xeng/1(data256_ready)
  Logical15/1 -> edge_detect3/1(in)
  Delay10/1 -> pack_xeng/2(data256_valid)
  Delay11/1 -> pack_xeng/3(data256)
  Delay12/1 -> pack_xeng/4(hdr_heap_id)
  Constant6/1 -> pack_xeng/5(hdr_heap_size)
  Delay14/1 -> pack_xeng/6(hdr_heap_offset)
  Delay15/1 -> pack_xeng/7(hdr_pkt_len_words)
  Delay16/1 -> pack_xeng/8(hdr5_0x1600_DIR)
  Gateway Out20/1 -> hdr_check1/4
  Gateway Out12/1 -> hdr_check1/1
  Gateway Out19/1 -> hdr_check1/3
  Gateway Out21/1 -> hdr_check1/5
  Gateway Out13/1 -> hdr_check1/2
  [valid_input] -> Gateway Out12/1
  [rb_done] -> Gateway Out13/1
  [end_of_vector] -> Gateway Out19/1
  [err] -> Gateway Out20/1
  [data_overflow] -> Gateway Out21/1
  [busy_pkt] -> Logical9/2
  Constant/1 -> Gateway Out8/1
  Constant4/1 -> Gateway Out14/1
  Convert3/1 -> Delay12/1
  [timestamp] -> Convert4/1
  [cnt_rst] -> vacc_monitor3/1(cnt_rst)
  vacc_monitor3/1(pkt_cnt) -> status/1(out_pkt_cnt)
  Delay6/1 -> edge_detect4/1(in)
  [eof_out] -> vacc_monitor3/2(eof)
  [err] -> vacc_monitor3/3(error)
  [data_overflow] -> vacc_monitor3/4(overflow)
  vacc_monitor3/2(error_cnt) -> status/2(out_align_err_cnt)
  vacc_monitor3/3(overflow_cnt) -> status/3(out_overflow_err_cnt)
